simulink model "CabinGuard_MATLAB_simulation"  (R2024a)
settings: Solver=ode4  StartTime=0.0  StopTime=45  FixedStep=0.01  RelTol=1e-3
undefined symbols (not defined in the file or in its folder): ca_a_comf, ca_a_lo, ca_absvel, ca_clear, ca_d0, ca_det, ca_edge, ca_ego_id, ca_go_phase, ca_hw, ca_jdn, ca_jup, ca_kfeas, ca_lka_in, ca_lka_out, ca_lw0, ca_min_shift, ca_plant, ca_psi0, ca_pv, ca_sys, ca_t_act, ca_v0, ca_vlat, ca_wn, ca_X0, ca_Y0, driving, matlabshared
libraries: simulink x102, drivingscenarioandsensors x5, autolibshared x2, mpcadaslib x1, slpidlib x1
(part 3 of 4)

== system CabinGuard_MATLAB_simulation/GNC/Control ==
  d : Inport
  e2 : Inport  Port=2
  kappa : Inport  Port=3
  vmeas : Inport  Port=4
  yref : Inport  Port=5
  ydot : Inport  Port=6
  vref : Inport  Port=7
  aref : Inport  Port=8
  act : Inport  Port=9
  up : Inport  Port=10
  lo : Inport  Port=11
  DevErr : Sum  Inputs=+-
  FF : Sum
  GwClamp : simulink/Discontinuities/Saturation Dynamic  OutMin=[]  OutMax=[]  OutDataTypeStr=Inherit: Same as second input  OutDataType=fixdt(1, 16)  OutScaling=2^-10  DoSatur=off
  HoldA : Constant  Value=-1.5
  HoldAnd : Logic  AllPortsSameDT=off  OutDataTypeStr=boolean
  HoldSw : Switch  Criteria=u2 ~= 0  SaturateOnIntegerOverflow=off  InputSameDT=off
  InDev : Gain  Gain=ca_lka_in
  InKap : Gain  Gain=ca_lka_in
  InYaw : Gain  Gain=ca_lka_in
  LKA : mpcadaslib/Lane Keeping Assist System  ModelType=Use vehicle parameters  VehicleMass=1500  VehicleYawInertia=2500  LengthToFront=1.2  LengthToRear=1.5  FrontTireStiffness=98100  RearTireStiffness=78480  EgoModelMatrixA=[-4.4021 ,-12.4603;1.3913,-5.1868]  EgoModelMatrixB=[24.1270;15.8609]  EgoModelMatrixC=[1,0;0,1]  InitialLongVel=15  TransportLag=ca_lka_lag  MinSteering=-0.1  umin_ext=off  MaxSteering=0.1  umax_ext=off  Ts=0.1  PredictionHorizon=10  ControllerBehavior=ca_lka_beh  suboptimal=off  maxiter=10  datatypeopt=double  optmode=off  trackmode=off
  OutSt : Gain  Gain=ca_lka_out
  Slow : simulink/Logic and Bit Operations/Compare To Constant  relop=<  const=0.3  OutDataTypeStr=boolean
  SpeedPID : slpidlib/PID Controller  Controller=PI  Form=Parallel  TimeDomain=Discrete-time  UseExternalTs=off  SampleTime=0.1  IntegratorMethod=Forward Euler  FilterMethod=Forward Euler  ControllerParametersSource=internal  P=1.2  I=0.25  UseKiTs=off  D=0  UseExternalDerivativeSource=off  N=100  UseFilter=on  TunerSelectOption=Transfer Function Based (PID Tuner App)  InitialConditionSource=internal  InitialConditionForIntegrator=0  InitialConditionForFilter=0  DifferentiatorICPrevScaledInput=0  ExternalReset=none  TrackingMode=off  Kt=1  LimitOutput=on  SatLimitsSource=internal  UpperSaturationLimit=2  LowerSaturationLimit=-9  LinearizeAsGain=on  AntiWindupMode=clamping  Kb=1  LimitIntegrator=off  UpperIntegratorSaturationLimit=inf  LowerIntegratorSaturationLimit=-inf  POutMin=[]  POutMax=[]  IOutMin=[]  IOutMax=[]  DOutMin=[]  DOutMax=[]  NOutMin=[]  NOutMax=[]  SumOutMin=[]  SumOutMax=[]  SaturationOutMin=[]  SaturationOutMax=[]  PParamMin=[]  PParamMax=[]  IParamMin=[]  IParamMax=[]  DParamMin=[]  DParamMax=[]  NParamMin=[]  NParamMax=[]  KbParamMin=[]  KbParamMax=[]  KtParamMin=[]  KtParamMax=[]  KbOutMin=[]  KbOutMax=[]  KtOutMin=[]  KtOutMax=[]  IntegratorOutMin=[]  IntegratorOutMax=[]  FilterOutMin=[]  FilterOutMax=[]  SumI1OutMin=[]  SumI1OutMax=[]  SumI2OutMin=[]  SumI2OutMax=[]  SumI3OutMin=[]  SumI3OutMax=[]  SumI4OutMin=[]  SumI4OutMax=[]  SumDOutMin=[]  SumDOutMax=[]  DifferentiatorOutMin=[]  DifferentiatorOutMax=[]  FilterDiffOutCoefMin=[]  FilterDiffOutCoefMax=[]  ReciprocalOutMin=[]  ReciprocalOutMax=[]  SumDenOutMin=[]  SumDenOutMax=[]  SumNumOutMin=[]  SumNumOutMax=[]  DivideOutMin=[]  DivideOutMax=[]  UdiffTsProdOutMin=[]  UdiffTsProdOutMax=[]  NTsProdOutMin=[]  NTsProdOutMax=[]  UintegralTsProdOutMin=[]  UintegralTsProdOutMax=[]  UngainTsProdOutMin=[]  UngainTsProdOutMax=[]  ClampingZeroOutDataTypeStr=Inherit: Inherit via back propagation  ClampingZeroOutMin=[]  ClampingZeroOutMax=[]  FilterDenConstantOutDataTypeStr=Inherit: Inherit via back propagation  FilterDenConstantOutMin=[]  FilterDenConstantOutMax=[]  PCopyOutDataTypeStr=Inherit: Inherit via back propagation  PCopyOutMin=[]  PCopyOutMax=[]  NCopyOutDataTypeStr=Inherit: Inherit via back propagation  NCopyOutMin=[]  NCopyOutMax=[]  IntegratorContinuousStateAttributes=''  IntegratorStateMustResolveToSignalObject=off  IntegratorRTWStateStorageClass=Auto  FilterContinuousStateAttributes=''  FilterStateMustResolveToSignalObject=off  FilterRTWStateStorageClass=Auto  ParallelPVariant=InternalParameters  IdealPVariant=Disabled  IVariant=InternalParameters  DVariant=Disabled  IntegratorVariant=Discrete  SatVariant=Enabled  AWVariant=DiscClampingParallel  PCopyVariant=Disabled  TRVariant=Disabled  FdbkBlocksVariant=Forward  IdealPFdbkVariant=Disabled  SatFdbkVariant=Disabled  DerivativeFilterVariant=Disabled  NVariant=Disabled  NCopyVariant=Disabled_SignalSpec  FilterICVariant=Disabled  IntegratorICVariant=InternalICs  ExternalResetVariant=Disabled  TRSumVariant=Passthrough  SumFdbkVariant=Disabled  SumVariant=Sum_PI  TsampFilterVariant=InternalTs  TsampNgainVariant=Passthrough  TsampIntegralVariant=Disabled_SignalSpec  ExternalSaturationOutDataTypeStr=Inherit: Same as second input  DerivativeSourceVariant=Disabled
  StSw : Switch  Threshold=0.5  SaturateOnIntegerOverflow=off  InputSameDT=off
  SteerLim : Saturate  UpperLimit=0.1  LowerLimit=-0.1
  StraightC : Constant  Value=0
  VErr : Sum  Inputs=+-
  VLka : Saturate  UpperLimit=40  LowerLimit=1
  VxeS : Saturate  UpperLimit=inf  LowerLimit=2
  YawErr : Sum  Inputs=+-
  YdDivV : Product  Inputs=*/
  dcmd : Outport
  acmd : Outport  Port=2
  wires:
  vmeas/1 -> StSw/2, VLka/1, VErr/2, VxeS/1, Slow/1
  VErr/1 -> SpeedPID/1
  Slow/1 -> HoldAnd/2
  OutSt/1 -> SteerLim/1
  vref/1 -> VErr/1
  ydot/1 -> YdDivV/1
  VxeS/1 -> YdDivV/2
  act/1 -> HoldAnd/1
  d/1 -> DevErr/1
  yref/1 -> DevErr/2
  e2/1 -> YawErr/1
  YdDivV/1 -> YawErr/2
  InDev/1 -> LKA/3
  HoldAnd/1 -> HoldSw/2
  SpeedPID/1 -> FF/1
  aref/1 -> FF/2
  kappa/1 -> InKap/1
  StraightC/1 -> StSw/3
  DevErr/1 -> InDev/1
  SteerLim/1 -> StSw/1
  YawErr/1 -> InYaw/1
  up/1 -> GwClamp/1
  lo/1 -> GwClamp/3
  FF/1 -> GwClamp/2
  InKap/1 -> LKA/1
  VLka/1 -> LKA/2
  InYaw/1 -> LKA/4
  LKA/1 -> OutSt/1
  HoldA/1 -> HoldSw/1
  GwClamp/1 -> HoldSw/3
  HoldSw/1 -> acmd/1
  StSw/1 -> dcmd/1

== system CabinGuard_MATLAB_simulation/GNC/Decision ==
  areq : Inport
  occ : Inport  Port=2
  vmeas : Inport  Port=3
  go : Inport  Port=4
  ActDbl : DataTypeConversion  OutDataTypeStr=double  SaturateOnIntegerOverflow=off  RndMeth=Floor
  Active : DataTypeConversion  OutDataTypeStr=boolean  SaturateOnIntegerOverflow=off  RndMeth=Floor
  Clear : Constant  Value=ca_clear
  Comf : Constant  Value=ca_a_comf
  CommitD : UnitDelay  SampleTime=0.1  HasFrameUpgradeWarning=on
  CommitDbl : DataTypeConversion  OutDataTypeStr=double  SaturateOnIntegerOverflow=off  RndMeth=Floor
  CommitOr : Logic  Operator=OR  AllPortsSameDT=off  OutDataTypeStr=boolean
  Edge : Constant  Value=ca_edge
  FeasCmp : RelationalOperator  OutDataTypeStr=boolean  RndMeth=Simplest  InputSameDT=off
  FeasDiv : Product  Inputs=*/
  FeasK : Gain  Gain=ca_kfeas*ca_vlat
  Go : Logic  Inputs=4  AllPortsSameDT=off  OutDataTypeStr=boolean
  MaxA : MinMax  Function=max  Inputs=2
  NegA : Gain  Gain=-1
  NotOcc : Logic  Operator=NOT  AllPortsSameDT=off  OutDataTypeStr=boolean
  ReqScaled : Gain  Gain=1.25
  SatA : Saturate  UpperLimit=8.5  LowerLimit=0
  Space : simulink/Logic and Bit Operations/Compare To Constant  relop=>=  const=ca_min_shift  OutDataTypeStr=boolean
  UNeg : Gain  Gain=-1
  UProd : Product  Inputs=**
  YshT : Sum  Inputs=+-
  ulat : Outport
  adem : Outport  Port=2
  act : Outport  Port=3
  yshT : Outport  Port=4
  commit : Outport  Port=5
  wires:
  go/1 -> Active/1
  SatA/1 -> FeasDiv/2, NegA/1
  vmeas/1 -> FeasK/1
  areq/1 -> ReqScaled/1
  CommitDbl/1 -> UProd/1, commit/1
  Clear/1 -> YshT/1
  Comf/1 -> MaxA/1
  Edge/1 -> YshT/2
  FeasCmp/1 -> Go/4
  Space/1 -> Go/2
  MaxA/1 -> SatA/1
  CommitOr/1 -> CommitD/1, CommitDbl/1
  ReqScaled/1 -> MaxA/2
  FeasK/1 -> FeasDiv/1
  FeasDiv/1 -> FeasCmp/1
  NegA/1 -> adem/1
  occ/1 -> NotOcc/1
  YshT/1 -> UProd/2, Space/1, FeasCmp/2, yshT/1
  Active/1 -> Go/1, ActDbl/1
  NotOcc/1 -> Go/3
  ActDbl/1 -> act/1
  UNeg/1 -> ulat/1
  Go/1 -> CommitOr/1
  CommitD/1 -> CommitOr/2
  UProd/1 -> UNeg/1

== system CabinGuard_MATLAB_simulation/GNC/Guidance ==
  adem : Inport
  ulat : Inport  Port=2
  go : Inport  Port=3
  ASw : Switch  Criteria=u2 ~= 0  SaturateOnIntegerOverflow=off  InputSameDT=off
  AZero : Constant  Value=0
  ActD : DataTypeConversion  OutDataTypeStr=double  SaturateOnIntegerOverflow=off  RndMeth=Floor
  Active : DataTypeConversion  OutDataTypeStr=boolean  SaturateOnIntegerOverflow=off  RndMeth=Floor
  ClampMax : Constant  Value=ca_a_lo
  Jerk : RateLimiter  RisingSlewLimit=ca_jup  FallingSlewLimit=-ca_jdn  SampleTimeMode=inherited
  LatRL : RateLimiter  RisingSlewLimit=ca_vlat  FallingSlewLimit=-ca_vlat  SampleTimeMode=inherited
  LcY : TransferFcn  Numerator=ca_wn^2  Denominator=[1 2*ca_wn ca_wn^2]
  LcYd : TransferFcn  Numerator=[ca_wn^2 0]  Denominator=[1 2*ca_wn ca_wn^2]
  LoIdle : Constant  Value=-6
  LoMax : MinMax  Function=max  Inputs=2
  LoSw : Switch  Criteria=u2 ~= 0  SaturateOnIntegerOverflow=off  InputSameDT=off
  UpAct : Constant  Value=0
  UpIdle : Constant  Value=2
  UpSw : Switch  Criteria=u2 ~= 0  SaturateOnIntegerOverflow=off  InputSameDT=off
  VRef : Integrator  InitialCondition=ca_v0  LimitOutput=on  LowerSaturationLimit=0
  yref : Outport
  ydot : Outport  Port=2
  vref : Outport  Port=3
  aref : Outport  Port=4
  act : Outport  Port=5
  actd : Outport  Port=6
  up : Outport  Port=7
  lo : Outport  Port=8
  wires:
  go/1 -> Active/1
  adem/1 -> ASw/1, LoMax/2
  ulat/1 -> LatRL/1
  LoIdle/1 -> LoSw/3
  LoMax/1 -> LoSw/1
  LatRL/1 -> LcYd/1, LcY/1
  LoSw/1 -> lo/1
  ClampMax/1 -> LoMax/1
  ASw/1 -> Jerk/1
  Active/1 -> UpSw/2, ASw/2, act/1, ActD/1, LoSw/2
  AZero/1 -> ASw/3
  UpAct/1 -> UpSw/1
  UpIdle/1 -> UpSw/3
  UpSw/1 -> up/1
  LcY/1 -> yref/1
  VRef/1 -> vref/1
  LcYd/1 -> ydot/1
  ActD/1 -> actd/1
  Jerk/1 -> VRef/1, aref/1

== system CabinGuard_MATLAB_simulation/GNC/Navigation ==
  Lanes : Inport
  vx : Inport  Port=2
  B1 : BusSelector  OutputSignals=LateralOffset,HeadingAngle,Curvature
  B2 : BusSelector  OutputSignals=LateralOffset,HeadingAngle,Curvature
  DSum : Sum  Inputs=+-
  FinAbs : Abs  SaturateOnIntegerOverflow=off
  FinCmp : simulink/Logic and Bit Operations/Compare To Constant  relop=<  const=1000  OutDataTypeStr=boolean
  FinSum : Sum  Inputs=+++
  GoodAnd : Logic  AllPortsSameDT=off  OutDataTypeStr=boolean
  H{1..4} (4 alike) : Switch  Criteria=u2 ~= 0  SaturateOnIntegerOverflow=off  InputSameDT=off
  Hd1 : UnitDelay  SampleTime=0.1  HasFrameUpgradeWarning=on
  Hd2 : UnitDelay  SampleTime=0.1  HasFrameUpgradeWarning=on
  Hd3 : UnitDelay  SampleTime=0.1  HasFrameUpgradeWarning=on
  Hd4 : UnitDelay  InitialCondition=ca_lw0  SampleTime=0.1  HasFrameUpgradeWarning=on
  JDiv : Product  Inputs=*/
  JMul : Product  Inputs=**
  JRnd : Rounding  Operator=round
  Jump : Sum  Inputs=+-
  LBS : BusSelector  OutputSignals=LaneBoundaries,NumLaneBoundaries
  Lane1 : Selector  IndexOptions=Index vector (dialog)  Indices=1  OutputSizes=1
  Lane2 : Selector  IndexOptions=Index vector (dialog)  Indices=2  OutputSizes=1
  Nd : UnitDelay  SampleTime=0.1  HasFrameUpgradeWarning=on
  Nsum : Sum
  PrevE1 : UnitDelay  SampleTime=0.1  HasFrameUpgradeWarning=on
  Valid : simulink/Logic and Bit Operations/Compare To Constant  relop=>=  const=2  OutDataTypeStr=boolean
  WsNoise : RandomNumber  Variance=0.0025  Seed=7  SampleTime=0.1
  WsSum : Sum
  WsZoh : ZeroOrderHold  SampleTime=0.1
  gCv : Gain  Gain=0.5*pi/180
  gHd : Gain  Gain=-0.5*pi/180
  gOff : Gain  Gain=-0.5
  sCv : Sum
  sHd : Sum
  sOff : Sum
  sWd : Sum  Inputs=+-
  e1 : Outport
  e2 : Outport  Port=2
  kappa : Outport  Port=3
  vmeas : Outport  Port=4
  d : Outport  Port=5
  wires:
  Lanes/1 -> LBS/1
  vx/1 -> WsSum/1
  Valid/1 -> GoodAnd/1
  Lane1/1 -> B1/1
  gCv/1 -> H3/1, FinSum/3
  LBS/1 -> Lane1/1, Lane2/1  "<LaneBoundaries>"
  sCv/1 -> gCv/1
  WsSum/1 -> WsZoh/1
  gOff/1 -> H1/1, FinSum/1
  sWd/1 -> H4/1
  WsNoise/1 -> WsSum/2
  Jump/1 -> JDiv/1
  WsZoh/1 -> vmeas/1
  PrevE1/1 -> Jump/2
  LBS/2 -> Valid/1  "<NumLaneBoundaries>"
  Lane2/1 -> B2/1
  B1/1 -> sWd/1, sOff/1  "<LateralOffset>"
  B1/2 -> sHd/1  "<HeadingAngle>"
  B1/3 -> sCv/1  "<Curvature>"
  B2/1 -> sWd/2, sOff/2  "<LateralOffset>"
  H4/1 -> Hd4/1
  B2/2 -> sHd/2  "<HeadingAngle>"
  Hd3/1 -> H3/3
  B2/3 -> sCv/2  "<Curvature>"
  sOff/1 -> gOff/1
  Nsum/1 -> DSum/2, Nd/1
  sHd/1 -> gHd/1
  gHd/1 -> H2/1, FinSum/2
  FinSum/1 -> FinAbs/1
  JDiv/1 -> JRnd/1
  FinAbs/1 -> FinCmp/1
  H3/1 -> kappa/1, Hd3/1
  FinCmp/1 -> GoodAnd/2
  Hd1/1 -> H1/3
  JMul/1 -> Nsum/1
  Hd4/1 -> JDiv/2, JMul/2, H4/3
  GoodAnd/1 -> H3/2, H2/2, H4/2, H1/2
  H2/1 -> Hd2/1, e2/1
  Hd2/1 -> H2/3
  H1/1 -> Hd1/1, PrevE1/1, e1/1, DSum/1, Jump/1
  DSum/1 -> d/1
  Nd/1 -> Nsum/2
  JRnd/1 -> JMul/1

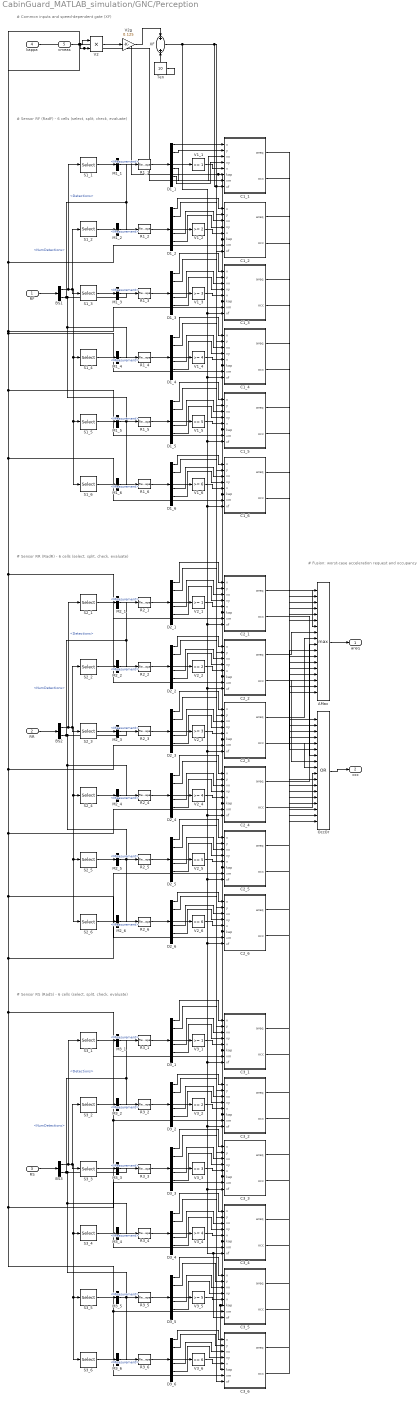
== system CabinGuard_MATLAB_simulation/GNC/Perception ==
  note: # Common inputs and speed-dependent gate (XF)
  note: # Sensor RF (RadF) - 6 cells (select, split, check, evaluate)
  note: # Sensor RR (RadR) - 6 cells (select, split, check, evaluate)
  note: # Sensor RS (RadS) - 6 cells (select, split, check, evaluate)
  note: # Fusion: worst-case acceleration request and occupancy
  RF : Inport
  RR : Inport  Port=2
  RS : Inport  Port=3
  kappa : Inport  Port=4
  vmeas : Inport  Port=5
  AMax : MinMax  Function=max  Inputs=18
  BS1 : BusSelector  OutputSignals=Detections,NumDetections
  BS2 : BusSelector  OutputSignals=Detections,NumDetections
  BS3 : BusSelector  OutputSignals=Detections,NumDetections
  C1_1 : Subsystem
  C1_2 : Subsystem
  C1_3 : Subsystem
  C1_4 : Subsystem
  C1_5 : Subsystem
  C1_6 : Subsystem
  C2_1 : Subsystem
  C2_2 : Subsystem
  C2_3 : Subsystem
  C2_4 : Subsystem
  C2_5 : Subsystem
  C2_6 : Subsystem
  C3_1 : Subsystem
  C3_2 : Subsystem
  C3_3 : Subsystem
  C3_4 : Subsystem
  C3_5 : Subsystem
  C3_6 : Subsystem
  D1_{1..6} (6 alike) : Demux  Outputs=6
  D2_{1..6} (6 alike) : Demux  Outputs=6
  D3_{1..6} (6 alike) : Demux  Outputs=6
  M1_{1..6} (6 alike) : BusSelector  OutputSignals=Measurement
  M2_{1..6} (6 alike) : BusSelector  OutputSignals=Measurement
  M3_{1..6} (6 alike) : BusSelector  OutputSignals=Measurement
  OccOr : Logic  Operator=OR  Inputs=18  AllPortsSameDT=off  OutDataTypeStr=boolean
  R1_{1..6} (6 alike) : Reshape
  R2_{1..6} (6 alike) : Reshape
  R3_{1..6} (6 alike) : Reshape
  S1_1 : Selector  IndexOptions=Index vector (dialog)  Indices=1  OutputSizes=1
  S1_2 : Selector  IndexOptions=Index vector (dialog)  Indices=2  OutputSizes=1
  S1_3 : Selector  IndexOptions=Index vector (dialog)  Indices=3  OutputSizes=1
  S1_4 : Selector  IndexOptions=Index vector (dialog)  Indices=4  OutputSizes=1
  S1_5 : Selector  IndexOptions=Index vector (dialog)  Indices=5  OutputSizes=1
  S1_6 : Selector  IndexOptions=Index vector (dialog)  Indices=6  OutputSizes=1
  S2_1 : Selector  IndexOptions=Index vector (dialog)  Indices=1  OutputSizes=1
  S2_2 : Selector  IndexOptions=Index vector (dialog)  Indices=2  OutputSizes=1
  S2_3 : Selector  IndexOptions=Index vector (dialog)  Indices=3  OutputSizes=1
  S2_4 : Selector  IndexOptions=Index vector (dialog)  Indices=4  OutputSizes=1
  S2_5 : Selector  IndexOptions=Index vector (dialog)  Indices=5  OutputSizes=1
  S2_6 : Selector  IndexOptions=Index vector (dialog)  Indices=6  OutputSizes=1
  S3_1 : Selector  IndexOptions=Index vector (dialog)  Indices=1  OutputSizes=1
  S3_2 : Selector  IndexOptions=Index vector (dialog)  Indices=2  OutputSizes=1
  S3_3 : Selector  IndexOptions=Index vector (dialog)  Indices=3  OutputSizes=1
  S3_4 : Selector  IndexOptions=Index vector (dialog)  Indices=4  OutputSizes=1
  S3_5 : Selector  IndexOptions=Index vector (dialog)  Indices=5  OutputSizes=1
  S3_6 : Selector  IndexOptions=Index vector (dialog)  Indices=6  OutputSizes=1
  Ten : Constant  Value=10
  V1_1 : simulink/Logic and Bit Operations/Compare To Constant  relop=>=  const=1  OutDataTypeStr=boolean
  V1_2 : simulink/Logic and Bit Operations/Compare To Constant  relop=>=  const=2  OutDataTypeStr=boolean
  V1_3 : simulink/Logic and Bit Operations/Compare To Constant  relop=>=  const=3  OutDataTypeStr=boolean
  V1_4 : simulink/Logic and Bit Operations/Compare To Constant  relop=>=  const=4  OutDataTypeStr=boolean
  V1_5 : simulink/Logic and Bit Operations/Compare To Constant  relop=>=  const=5  OutDataTypeStr=boolean
  V1_6 : simulink/Logic and Bit Operations/Compare To Constant  relop=>=  const=6  OutDataTypeStr=boolean
  V2 : Product  Inputs=**
  V2_1 : simulink/Logic and Bit Operations/Compare To Constant  relop=>=  const=1  OutDataTypeStr=boolean
  V2_2 : simulink/Logic and Bit Operations/Compare To Constant  relop=>=  const=2  OutDataTypeStr=boolean
  V2_3 : simulink/Logic and Bit Operations/Compare To Constant  relop=>=  const=3  OutDataTypeStr=boolean
  V2_4 : simulink/Logic and Bit Operations/Compare To Constant  relop=>=  const=4  OutDataTypeStr=boolean
  V2_5 : simulink/Logic and Bit Operations/Compare To Constant  relop=>=  const=5  OutDataTypeStr=boolean
  V2_6 : simulink/Logic and Bit Operations/Compare To Constant  relop=>=  const=6  OutDataTypeStr=boolean
  V2g : Gain  Gain=0.125
  V3_1 : simulink/Logic and Bit Operations/Compare To Constant  relop=>=  const=1  OutDataTypeStr=boolean
  V3_2 : simulink/Logic and Bit Operations/Compare To Constant  relop=>=  const=2  OutDataTypeStr=boolean
  V3_3 : simulink/Logic and Bit Operations/Compare To Constant  relop=>=  const=3  OutDataTypeStr=boolean
  V3_4 : simulink/Logic and Bit Operations/Compare To Constant  relop=>=  const=4  OutDataTypeStr=boolean
  V3_5 : simulink/Logic and Bit Operations/Compare To Constant  relop=>=  const=5  OutDataTypeStr=boolean
  V3_6 : simulink/Logic and Bit Operations/Compare To Constant  relop=>=  const=6  OutDataTypeStr=boolean
  XF : Sum
  areq : Outport
  occ : Outport  Port=2
  wires:
  vmeas/1 -> C3_5/7(vm), C3_6/7(vm), C3_3/7(vm), C3_1/7(vm), C2_5/7(vm), C2_4/7(vm), C2_3/7(vm), C2_1/7(vm), C1_5/7(vm), C1_3/7(vm), C1_2/7(vm), C1_1/7(vm), V2/2, V2/1, C3_2/7(vm), C3_4/7(vm), C2_6/7(vm), C2_2/7(vm), C1_6/7(vm), C1_4/7(vm)
  V2/1 -> V2g/1
  V2g/1 -> XF/1
  Ten/1 -> XF/2
  RF/1 -> BS1/1
  BS1/1 -> S1_2/1, S1_3/1, S1_4/1, S1_5/1, S1_6/1, S1_1/1  "<Detections>"
  S1_1/1 -> M1_1/1
  M1_1/1 -> R1_1/1  "<Measurement>"
  R1_1/1 -> D1_1/1
  BS1/2 -> V1_3/1, V1_5/1, V1_6/1, V1_4/1, V1_1/1, V1_2/1  "<NumDetections>"
  D1_1/1 -> C1_1/1(x)
  D1_1/2 -> C1_1/2(y)
  D1_1/4 -> C1_1/3(vx)
  D1_1/5 -> C1_1/4(vy)
  V1_1/1 -> C1_1/5(v)
  kappa/1 -> C3_6/6(kap), C3_5/6(kap), C3_4/6(kap), C3_3/6(kap), C3_2/6(kap), C3_1/6(kap), C2_6/6(kap), C2_5/6(kap), C2_4/6(kap), C2_3/6(kap), C2_2/6(kap), C2_1/6(kap), C1_6/6(kap), C1_5/6(kap), C1_4/6(kap), C1_3/6(kap), C1_2/6(kap), C1_1/6(kap)
  XF/1 -> C3_5/8(xf), C3_4/8(xf), C3_3/8(xf), C3_2/8(xf), C3_1/8(xf), C2_6/8(xf), C2_5/8(xf), C2_4/8(xf), C2_3/8(xf), C2_2/8(xf), C2_1/8(xf), C1_6/8(xf), C1_5/8(xf), C1_4/8(xf), C1_3/8(xf), C1_1/8(xf), C1_2/8(xf), C3_6/8(xf)
  C1_1/1(areq) -> AMax/1
  C1_1/2(occ) -> OccOr/1
  S1_2/1 -> M1_2/1
  M1_2/1 -> R1_2/1  "<Measurement>"
  R1_2/1 -> D1_2/1
  D1_2/1 -> C1_2/1(x)
  D1_2/2 -> C1_2/2(y)
  D1_2/4 -> C1_2/3(vx)
  D1_2/5 -> C1_2/4(vy)
  V1_2/1 -> C1_2/5(v)
  C1_2/1(areq) -> AMax/2
  C1_2/2(occ) -> OccOr/2
  S1_3/1 -> M1_3/1
  M1_3/1 -> R1_3/1  "<Measurement>"
  R1_3/1 -> D1_3/1
  D1_3/1 -> C1_3/1(x)
  D1_3/2 -> C1_3/2(y)
  D1_3/4 -> C1_3/3(vx)
  D1_3/5 -> C1_3/4(vy)
  V1_3/1 -> C1_3/5(v)
  C1_3/1(areq) -> AMax/3
  C1_3/2(occ) -> OccOr/3
  S1_4/1 -> M1_4/1
  M1_4/1 -> R1_4/1  "<Measurement>"
  R1_4/1 -> D1_4/1
  D1_4/1 -> C1_4/1(x)
  D1_4/2 -> C1_4/2(y)
  D1_4/4 -> C1_4/3(vx)
  D1_4/5 -> C1_4/4(vy)
  V1_4/1 -> C1_4/5(v)
  C1_4/1(areq) -> AMax/4
  C1_4/2(occ) -> OccOr/4
  S1_5/1 -> M1_5/1
  M1_5/1 -> R1_5/1  "<Measurement>"
  R1_5/1 -> D1_5/1
  D1_5/1 -> C1_5/1(x)
  D1_5/2 -> C1_5/2(y)
  D1_5/4 -> C1_5/3(vx)
  D1_5/5 -> C1_5/4(vy)
  V1_5/1 -> C1_5/5(v)
  C1_5/1(areq) -> AMax/5
  C1_5/2(occ) -> OccOr/5
  S1_6/1 -> M1_6/1
  M1_6/1 -> R1_6/1  "<Measurement>"
  R1_6/1 -> D1_6/1
  D1_6/1 -> C1_6/1(x)
  D1_6/2 -> C1_6/2(y)
  D1_6/4 -> C1_6/3(vx)
  D1_6/5 -> C1_6/4(vy)
  V1_6/1 -> C1_6/5(v)
  C1_6/1(areq) -> AMax/6
  C1_6/2(occ) -> OccOr/6
  RR/1 -> BS2/1
  BS2/1 -> S2_2/1, S2_3/1, S2_4/1, S2_5/1, S2_6/1, S2_1/1  "<Detections>"
  S2_1/1 -> M2_1/1
  M2_1/1 -> R2_1/1  "<Measurement>"
  R2_1/1 -> D2_1/1
  BS2/2 -> V2_3/1, V2_5/1, V2_6/1, V2_4/1, V2_1/1, V2_2/1  "<NumDetections>"
  D2_1/1 -> C2_1/1(x)
  D2_1/2 -> C2_1/2(y)
  D2_1/4 -> C2_1/3(vx)
  D2_1/5 -> C2_1/4(vy)
  V2_1/1 -> C2_1/5(v)
  C2_1/1(areq) -> AMax/7
  C2_1/2(occ) -> OccOr/7
  S2_2/1 -> M2_2/1
  M2_2/1 -> R2_2/1  "<Measurement>"
  R2_2/1 -> D2_2/1
  D2_2/1 -> C2_2/1(x)
  D2_2/2 -> C2_2/2(y)
  D2_2/4 -> C2_2/3(vx)
  D2_2/5 -> C2_2/4(vy)
  V2_2/1 -> C2_2/5(v)
  C2_2/1(areq) -> AMax/8
  C2_2/2(occ) -> OccOr/8
  S2_3/1 -> M2_3/1
  M2_3/1 -> R2_3/1  "<Measurement>"
  R2_3/1 -> D2_3/1
  D2_3/1 -> C2_3/1(x)
  D2_3/2 -> C2_3/2(y)
  D2_3/4 -> C2_3/3(vx)
  D2_3/5 -> C2_3/4(vy)
  V2_3/1 -> C2_3/5(v)
  C2_3/1(areq) -> AMax/9
  C2_3/2(occ) -> OccOr/9
  S2_4/1 -> M2_4/1
  M2_4/1 -> R2_4/1  "<Measurement>"
  R2_4/1 -> D2_4/1
  D2_4/1 -> C2_4/1(x)
  D2_4/2 -> C2_4/2(y)
  D2_4/4 -> C2_4/3(vx)
  D2_4/5 -> C2_4/4(vy)
  V2_4/1 -> C2_4/5(v)
  C2_4/1(areq) -> AMax/10
  C2_4/2(occ) -> OccOr/10
  S2_5/1 -> M2_5/1
  M2_5/1 -> R2_5/1  "<Measurement>"
  R2_5/1 -> D2_5/1
  D2_5/1 -> C2_5/1(x)
  D2_5/2 -> C2_5/2(y)
  D2_5/4 -> C2_5/3(vx)
  D2_5/5 -> C2_5/4(vy)
  V2_5/1 -> C2_5/5(v)
  C2_5/1(areq) -> AMax/11
  C2_5/2(occ) -> OccOr/11
  S2_6/1 -> M2_6/1
  M2_6/1 -> R2_6/1  "<Measurement>"
  R2_6/1 -> D2_6/1
  D2_6/1 -> C2_6/1(x)
  D2_6/2 -> C2_6/2(y)
  D2_6/4 -> C2_6/3(vx)
  D2_6/5 -> C2_6/4(vy)
  V2_6/1 -> C2_6/5(v)
  C2_6/1(areq) -> AMax/12
  C2_6/2(occ) -> OccOr/12
  RS/1 -> BS3/1
  BS3/1 -> S3_2/1, S3_3/1, S3_4/1, S3_5/1, S3_6/1, S3_1/1  "<Detections>"
  S3_1/1 -> M3_1/1
  M3_1/1 -> R3_1/1  "<Measurement>"
  R3_1/1 -> D3_1/1
  BS3/2 -> V3_3/1, V3_5/1, V3_6/1, V3_4/1, V3_1/1, V3_2/1  "<NumDetections>"
  D3_1/1 -> C3_1/1(x)
  D3_1/2 -> C3_1/2(y)
  D3_1/4 -> C3_1/3(vx)
  D3_1/5 -> C3_1/4(vy)
  V3_1/1 -> C3_1/5(v)
  C3_1/1(areq) -> AMax/13
  C3_1/2(occ) -> OccOr/13
  S3_2/1 -> M3_2/1
  M3_2/1 -> R3_2/1  "<Measurement>"
  R3_2/1 -> D3_2/1
  D3_2/1 -> C3_2/1(x)
  D3_2/2 -> C3_2/2(y)
  D3_2/4 -> C3_2/3(vx)
  D3_2/5 -> C3_2/4(vy)
  V3_2/1 -> C3_2/5(v)
  C3_2/1(areq) -> AMax/14
  C3_2/2(occ) -> OccOr/14
  S3_3/1 -> M3_3/1
  M3_3/1 -> R3_3/1  "<Measurement>"
  R3_3/1 -> D3_3/1
  D3_3/1 -> C3_3/1(x)
  D3_3/2 -> C3_3/2(y)
  D3_3/4 -> C3_3/3(vx)
  D3_3/5 -> C3_3/4(vy)
  V3_3/1 -> C3_3/5(v)
  C3_3/1(areq) -> AMax/15
  C3_3/2(occ) -> OccOr/15
  S3_4/1 -> M3_4/1
  M3_4/1 -> R3_4/1  "<Measurement>"
  R3_4/1 -> D3_4/1
  D3_4/1 -> C3_4/1(x)
  D3_4/2 -> C3_4/2(y)
  D3_4/4 -> C3_4/3(vx)
  D3_4/5 -> C3_4/4(vy)
  V3_4/1 -> C3_4/5(v)
  C3_4/1(areq) -> AMax/16
  C3_4/2(occ) -> OccOr/16
  S3_5/1 -> M3_5/1
  M3_5/1 -> R3_5/1  "<Measurement>"
  R3_5/1 -> D3_5/1
  D3_5/1 -> C3_5/1(x)
  D3_5/2 -> C3_5/2(y)
  D3_5/4 -> C3_5/3(vx)
  D3_5/5 -> C3_5/4(vy)
  V3_5/1 -> C3_5/5(v)
  C3_5/1(areq) -> AMax/17
  C3_5/2(occ) -> OccOr/17
  S3_6/1 -> M3_6/1
  M3_6/1 -> R3_6/1  "<Measurement>"
  R3_6/1 -> D3_6/1
  D3_6/1 -> C3_6/1(x)
  D3_6/2 -> C3_6/2(y)
  D3_6/4 -> C3_6/3(vx)
  D3_6/5 -> C3_6/4(vy)
  V3_6/1 -> C3_6/5(v)
  C3_6/1(areq) -> AMax/18
  C3_6/2(occ) -> OccOr/18
  AMax/1 -> areq/1
  OccOr/1 -> occ/1

== system CabinGuard_MATLAB_simulation/Vehicle/LBody ==
  FwF : Inport
  FwR : Inport  Port=2
  Grade : Inport  Port=3
  Wind : Inport  Port=4
  HoldIn : Inport  Port=5
  Brk : simulink/Logic and Bit Operations/Compare To Constant  relop=>  const=0.5  OutDataTypeStr=boolean
  CF : Constant  Value=4087.5
  CR : Constant  Value=3270
  Fsum : Sum
  HAnd : Logic  AllPortsSameDT=off  OutDataTypeStr=boolean
  HSw : Switch  Criteria=u2 ~= 0  SaturateOnIntegerOverflow=off  InputSameDT=off
  Hold : Gain  Gain=-20
  InvM : Gain  Gain=0.0006666666667
  Ix : Integrator  InitialCondition=ca_v0  LimitOutput=on  LowerSaturationLimit=0
  Kd : Gain  Gain=0.42175
  KhF : Gain  Gain=-152.7777778
  KhR : Gain  Gain=152.7777778
  Net : Sum  Inputs=+-
  Pitch : TransferFcn  Numerator=1  Denominator=[0.15 1]
  SF : Sum
  SR : Sum
  Slow : simulink/Logic and Bit Operations/Compare To Constant  relop=<  const=0.4  OutDataTypeStr=boolean
  TG : Terminator
  TW : Terminator
  V2 : Product
  Z : Constant  Value=0
  Info : Outport
  xdot : Outport  Port=2
  FzF : Outport  Port=3
  FzR : Outport  Port=4
  wires:
  Kd/1 -> Net/2
  V2/1 -> Kd/1
  HoldIn/1 -> Brk/1
  Grade/1 -> TG/1
  Slow/1 -> HAnd/1
  FwF/1 -> Fsum/1
  Wind/1 -> TW/1
  Z/1 -> Info/1
  InvM/1 -> HSw/3, Pitch/1
  FwR/1 -> Fsum/2
  Fsum/1 -> Net/1
  KhF/1 -> SF/1
  Brk/1 -> HAnd/2
  Net/1 -> InvM/1
  Ix/1 -> V2/1, Slow/1, Hold/1, xdot/1, V2/2
  HAnd/1 -> HSw/2
  Hold/1 -> HSw/1
  Pitch/1 -> KhF/1, KhR/1
  HSw/1 -> Ix/1
  CR/1 -> SR/2
  KhR/1 -> SR/1
  CF/1 -> SF/2
  SR/1 -> FzR/1
  SF/1 -> FzF/1

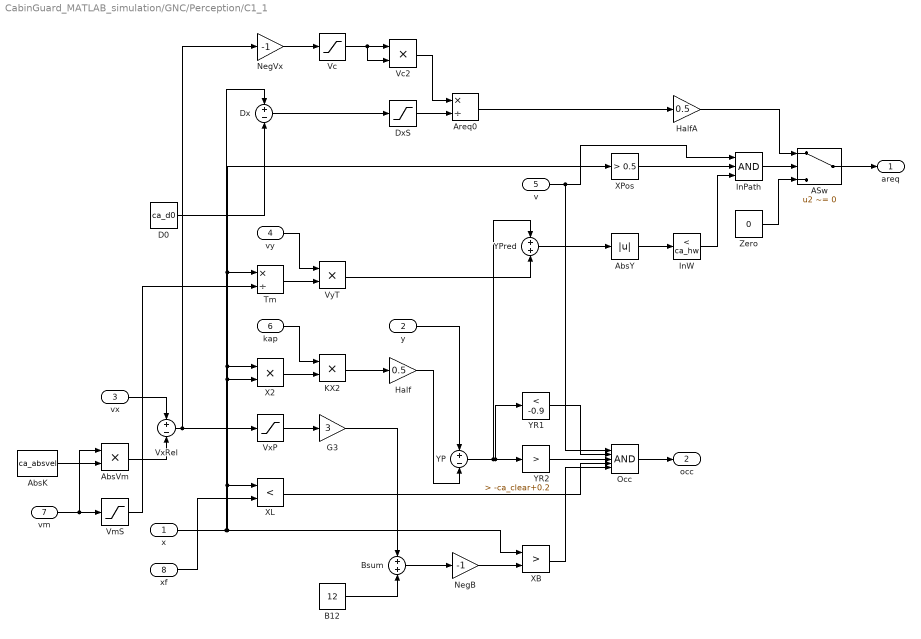
== system CabinGuard_MATLAB_simulation/GNC/Perception/C1_1 ==
  x : Inport
  y : Inport  Port=2
  vx : Inport  Port=3
  vy : Inport  Port=4
  v : Inport  Port=5
  kap : Inport  Port=6
  vm : Inport  Port=7
  xf : Inport  Port=8
  ASw : Switch  Criteria=u2 ~= 0  SaturateOnIntegerOverflow=off  InputSameDT=off
  AbsK : Constant  Value=ca_absvel
  AbsVm : Product  Inputs=**
  AbsY : Abs  SaturateOnIntegerOverflow=off
  Areq0 : Product  Inputs=*/
  B12 : Constant  Value=12
  Bsum : Sum
  D0 : Constant  Value=ca_d0
  Dx : Sum  Inputs=+-
  DxS : Saturate  UpperLimit=inf  LowerLimit=0.5
  G3 : Gain  Gain=3
  Half : Gain  Gain=0.5
  HalfA : Gain  Gain=0.5
  InPath : Logic  Inputs=3  AllPortsSameDT=off  OutDataTypeStr=boolean
  InW : simulink/Logic and Bit Operations/Compare To Constant  relop=<  const=ca_hw  OutDataTypeStr=boolean
  KX2 : Product  Inputs=**
  NegB : Gain  Gain=-1
  NegVx : Gain  Gain=-1
  Occ : Logic  Inputs=5  AllPortsSameDT=off  OutDataTypeStr=boolean
  Tm : Product  Inputs=*/
  Vc : Saturate  UpperLimit=inf  LowerLimit=0
  Vc2 : Product  Inputs=**
  VmS : Saturate  UpperLimit=inf  LowerLimit=1
  VxP : Saturate  UpperLimit=inf  LowerLimit=0
  VxRel : Sum  Inputs=+-
  VyT : Product  Inputs=**
  X2 : Product  Inputs=**
  XB : RelationalOperator  Operator=>  OutDataTypeStr=boolean  RndMeth=Simplest  InputSameDT=off
  XL : RelationalOperator  Operator=<  OutDataTypeStr=boolean  RndMeth=Simplest  InputSameDT=off
  XPos : simulink/Logic and Bit Operations/Compare To Constant  relop=>  const=0.5  OutDataTypeStr=boolean
  YP : Sum  Inputs=+-
  YPred : Sum
  YR1 : simulink/Logic and Bit Operations/Compare To Constant  relop=<  const=-0.9  OutDataTypeStr=boolean
  YR2 : simulink/Logic and Bit Operations/Compare To Constant  relop=>  const=-ca_clear+0.2  OutDataTypeStr=boolean
  Zero : Constant  Value=0
  areq : Outport
  occ : Outport  Port=2
  wires:
  Tm/1 -> VyT/2
  AbsK/1 -> AbsVm/2
  vx/1 -> VxRel/1
  InPath/1 -> ASw/2
  vm/1 -> AbsVm/1, VmS/1
  AbsVm/1 -> VxRel/2
  NegB/1 -> XB/2
  VmS/1 -> Tm/2
  x/1 -> Tm/1, XPos/1, X2/1, X2/2, XL/1, XB/1, Dx/1
  D0/1 -> Dx/2
  VxRel/1 -> VxP/1, NegVx/1
  Bsum/1 -> NegB/1
  xf/1 -> XL/2
  VxP/1 -> G3/1
  kap/1 -> KX2/1
  NegVx/1 -> Vc/1
  Dx/1 -> DxS/1
  vy/1 -> VyT/1
  X2/1 -> KX2/2
  XL/1 -> Occ/4
  InW/1 -> InPath/3
  Vc/1 -> Vc2/2, Vc2/1
  VyT/1 -> YPred/2
  AbsY/1 -> InW/1
  Vc2/1 -> Areq0/1
  KX2/1 -> Half/1
  y/1 -> YP/1
  G3/1 -> Bsum/1
  B12/1 -> Bsum/2
  DxS/1 -> Areq0/2
  Half/1 -> YP/2
  Areq0/1 -> HalfA/1
  YP/1 -> YR2/1, YR1/1, YPred/1
  HalfA/1 -> ASw/1
  v/1 -> InPath/1, Occ/1
  YPred/1 -> AbsY/1
  YR1/1 -> Occ/2
  YR2/1 -> Occ/3
  XB/1 -> Occ/5
  XPos/1 -> InPath/2
  Occ/1 -> occ/1
  Zero/1 -> ASw/3
  ASw/1 -> areq/1

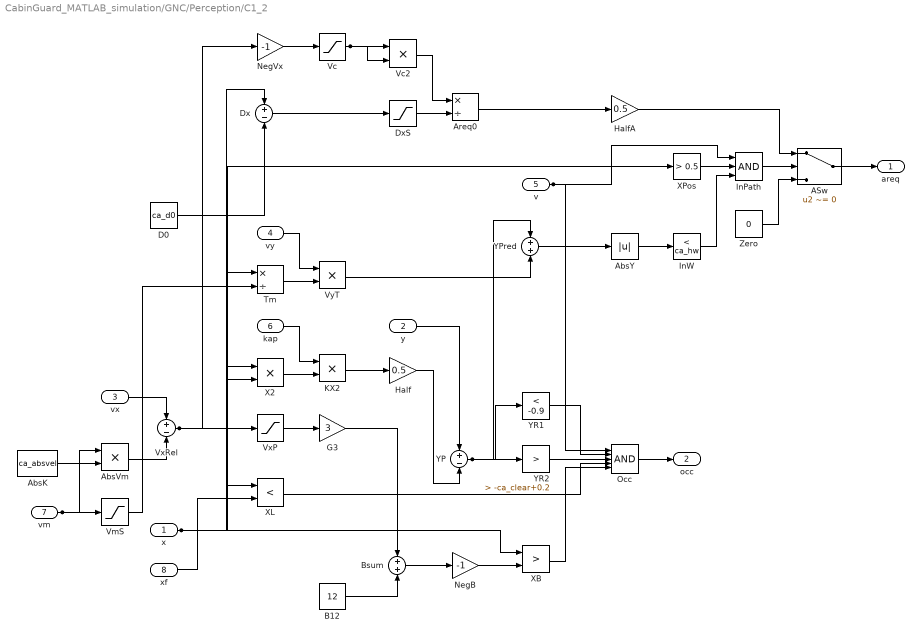
== system CabinGuard_MATLAB_simulation/GNC/Perception/C1_2 ==
  x : Inport
  y : Inport  Port=2
  vx : Inport  Port=3
  vy : Inport  Port=4
  v : Inport  Port=5
  kap : Inport  Port=6
  vm : Inport  Port=7
  xf : Inport  Port=8
  ASw : Switch  Criteria=u2 ~= 0  SaturateOnIntegerOverflow=off  InputSameDT=off
  AbsK : Constant  Value=ca_absvel
  AbsVm : Product  Inputs=**
  AbsY : Abs  SaturateOnIntegerOverflow=off
  Areq0 : Product  Inputs=*/
  B12 : Constant  Value=12
  Bsum : Sum
  D0 : Constant  Value=ca_d0
  Dx : Sum  Inputs=+-
  DxS : Saturate  UpperLimit=inf  LowerLimit=0.5
  G3 : Gain  Gain=3
  Half : Gain  Gain=0.5
  HalfA : Gain  Gain=0.5
  InPath : Logic  Inputs=3  AllPortsSameDT=off  OutDataTypeStr=boolean
  InW : simulink/Logic and Bit Operations/Compare To Constant  relop=<  const=ca_hw  OutDataTypeStr=boolean
  KX2 : Product  Inputs=**
  NegB : Gain  Gain=-1
  NegVx : Gain  Gain=-1
  Occ : Logic  Inputs=5  AllPortsSameDT=off  OutDataTypeStr=boolean
  Tm : Product  Inputs=*/
  Vc : Saturate  UpperLimit=inf  LowerLimit=0
  Vc2 : Product  Inputs=**
  VmS : Saturate  UpperLimit=inf  LowerLimit=1
  VxP : Saturate  UpperLimit=inf  LowerLimit=0
  VxRel : Sum  Inputs=+-
  VyT : Product  Inputs=**
  X2 : Product  Inputs=**
  XB : RelationalOperator  Operator=>  OutDataTypeStr=boolean  RndMeth=Simplest  InputSameDT=off
  XL : RelationalOperator  Operator=<  OutDataTypeStr=boolean  RndMeth=Simplest  InputSameDT=off
  XPos : simulink/Logic and Bit Operations/Compare To Constant  relop=>  const=0.5  OutDataTypeStr=boolean
  YP : Sum  Inputs=+-
  YPred : Sum
  YR1 : simulink/Logic and Bit Operations/Compare To Constant  relop=<  const=-0.9  OutDataTypeStr=boolean
  YR2 : simulink/Logic and Bit Operations/Compare To Constant  relop=>  const=-ca_clear+0.2  OutDataTypeStr=boolean
  Zero : Constant  Value=0
  areq : Outport
  occ : Outport  Port=2
  wires:
  AbsK/1 -> AbsVm/2
  Zero/1 -> ASw/3
  Areq0/1 -> HalfA/1
  D0/1 -> Dx/2
  HalfA/1 -> ASw/1
  YPred/1 -> AbsY/1
  vx/1 -> VxRel/1
  AbsVm/1 -> VxRel/2
  vm/1 -> AbsVm/1, VmS/1
  VmS/1 -> Tm/2
  xf/1 -> XL/2
  VxRel/1 -> VxP/1, NegVx/1
  AbsY/1 -> InW/1
  x/1 -> XB/1, XPos/1, XL/1, Tm/1, Dx/1, X2/2, X2/1
  G3/1 -> Bsum/1
  NegVx/1 -> Vc/1
  InPath/1 -> ASw/2
  Dx/1 -> DxS/1
  vy/1 -> VyT/1
  Tm/1 -> VyT/2
  kap/1 -> KX2/1
  Occ/1 -> occ/1
  X2/1 -> KX2/2
  VxP/1 -> G3/1
  XL/1 -> Occ/4
  Vc/1 -> Vc2/2, Vc2/1
  VyT/1 -> YPred/2
  KX2/1 -> Half/1
  B12/1 -> Bsum/2
  Vc2/1 -> Areq0/1
  NegB/1 -> XB/2
  y/1 -> YP/1
  DxS/1 -> Areq0/2
  Half/1 -> YP/2
  Bsum/1 -> NegB/1
  YP/1 -> YPred/1, YR1/1, YR2/1
  v/1 -> InPath/1, Occ/1
  YR1/1 -> Occ/2
  YR2/1 -> Occ/3
  XB/1 -> Occ/5
  XPos/1 -> InPath/2
  InW/1 -> InPath/3
  ASw/1 -> areq/1

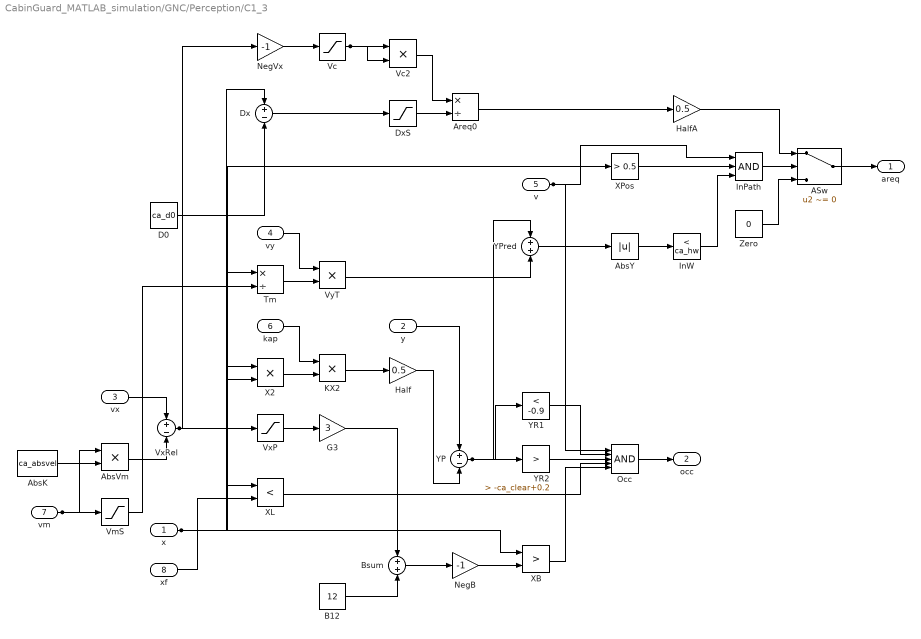
== system CabinGuard_MATLAB_simulation/GNC/Perception/C1_3 ==
  x : Inport
  y : Inport  Port=2
  vx : Inport  Port=3
  vy : Inport  Port=4
  v : Inport  Port=5
  kap : Inport  Port=6
  vm : Inport  Port=7
  xf : Inport  Port=8
  ASw : Switch  Criteria=u2 ~= 0  SaturateOnIntegerOverflow=off  InputSameDT=off
  AbsK : Constant  Value=ca_absvel
  AbsVm : Product  Inputs=**
  AbsY : Abs  SaturateOnIntegerOverflow=off
  Areq0 : Product  Inputs=*/
  B12 : Constant  Value=12
  Bsum : Sum
  D0 : Constant  Value=ca_d0
  Dx : Sum  Inputs=+-
  DxS : Saturate  UpperLimit=inf  LowerLimit=0.5
  G3 : Gain  Gain=3
  Half : Gain  Gain=0.5
  HalfA : Gain  Gain=0.5
  InPath : Logic  Inputs=3  AllPortsSameDT=off  OutDataTypeStr=boolean
  InW : simulink/Logic and Bit Operations/Compare To Constant  relop=<  const=ca_hw  OutDataTypeStr=boolean
  KX2 : Product  Inputs=**
  NegB : Gain  Gain=-1
  NegVx : Gain  Gain=-1
  Occ : Logic  Inputs=5  AllPortsSameDT=off  OutDataTypeStr=boolean
  Tm : Product  Inputs=*/
  Vc : Saturate  UpperLimit=inf  LowerLimit=0
  Vc2 : Product  Inputs=**
  VmS : Saturate  UpperLimit=inf  LowerLimit=1
  VxP : Saturate  UpperLimit=inf  LowerLimit=0
  VxRel : Sum  Inputs=+-
  VyT : Product  Inputs=**
  X2 : Product  Inputs=**
  XB : RelationalOperator  Operator=>  OutDataTypeStr=boolean  RndMeth=Simplest  InputSameDT=off
  XL : RelationalOperator  Operator=<  OutDataTypeStr=boolean  RndMeth=Simplest  InputSameDT=off
  XPos : simulink/Logic and Bit Operations/Compare To Constant  relop=>  const=0.5  OutDataTypeStr=boolean
  YP : Sum  Inputs=+-
  YPred : Sum
  YR1 : simulink/Logic and Bit Operations/Compare To Constant  relop=<  const=-0.9  OutDataTypeStr=boolean
  YR2 : simulink/Logic and Bit Operations/Compare To Constant  relop=>  const=-ca_clear+0.2  OutDataTypeStr=boolean
  Zero : Constant  Value=0
  areq : Outport
  occ : Outport  Port=2
  wires:
  AbsK/1 -> AbsVm/2
  AbsY/1 -> InW/1
  vx/1 -> VxRel/1
  vm/1 -> AbsVm/1, VmS/1
  AbsVm/1 -> VxRel/2
  VmS/1 -> Tm/2
  x/1 -> XB/1, XPos/1, Tm/1, Dx/1, X2/2, XL/1, X2/1
  D0/1 -> Dx/2
  VxRel/1 -> VxP/1, NegVx/1
  Bsum/1 -> NegB/1
  xf/1 -> XL/2
  NegVx/1 -> Vc/1
  YR1/1 -> Occ/2
  Dx/1 -> DxS/1
  vy/1 -> VyT/1
  Tm/1 -> VyT/2
  XB/1 -> Occ/5
  kap/1 -> KX2/1
  X2/1 -> KX2/2
  VxP/1 -> G3/1
  XL/1 -> Occ/4
  Vc/1 -> Vc2/2, Vc2/1
  VyT/1 -> YPred/2
  KX2/1 -> Half/1
  y/1 -> YP/1
  G3/1 -> Bsum/1
  B12/1 -> Bsum/2
  Vc2/1 -> Areq0/1
  DxS/1 -> Areq0/2
  Half/1 -> YP/2
  Areq0/1 -> HalfA/1
  YP/1 -> YPred/1, YR2/1, YR1/1
  NegB/1 -> XB/2
  HalfA/1 -> ASw/1
  v/1 -> InPath/1, Occ/1
  YPred/1 -> AbsY/1
  YR2/1 -> Occ/3
  XPos/1 -> InPath/2
  Occ/1 -> occ/1
  InW/1 -> InPath/3
  InPath/1 -> ASw/2
  Zero/1 -> ASw/3
  ASw/1 -> areq/1

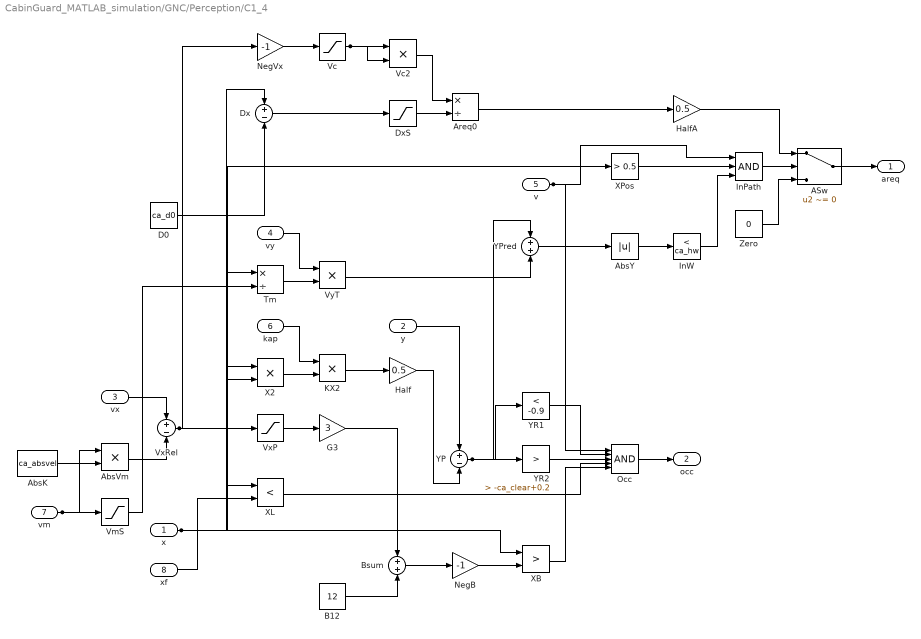
== system CabinGuard_MATLAB_simulation/GNC/Perception/C1_4 ==
  x : Inport
  y : Inport  Port=2
  vx : Inport  Port=3
  vy : Inport  Port=4
  v : Inport  Port=5
  kap : Inport  Port=6
  vm : Inport  Port=7
  xf : Inport  Port=8
  ASw : Switch  Criteria=u2 ~= 0  SaturateOnIntegerOverflow=off  InputSameDT=off
  AbsK : Constant  Value=ca_absvel
  AbsVm : Product  Inputs=**
  AbsY : Abs  SaturateOnIntegerOverflow=off
  Areq0 : Product  Inputs=*/
  B12 : Constant  Value=12
  Bsum : Sum
  D0 : Constant  Value=ca_d0
  Dx : Sum  Inputs=+-
  DxS : Saturate  UpperLimit=inf  LowerLimit=0.5
  G3 : Gain  Gain=3
  Half : Gain  Gain=0.5
  HalfA : Gain  Gain=0.5
  InPath : Logic  Inputs=3  AllPortsSameDT=off  OutDataTypeStr=boolean
  InW : simulink/Logic and Bit Operations/Compare To Constant  relop=<  const=ca_hw  OutDataTypeStr=boolean
  KX2 : Product  Inputs=**
  NegB : Gain  Gain=-1
  NegVx : Gain  Gain=-1
  Occ : Logic  Inputs=5  AllPortsSameDT=off  OutDataTypeStr=boolean
  Tm : Product  Inputs=*/
  Vc : Saturate  UpperLimit=inf  LowerLimit=0
  Vc2 : Product  Inputs=**
  VmS : Saturate  UpperLimit=inf  LowerLimit=1
  VxP : Saturate  UpperLimit=inf  LowerLimit=0
  VxRel : Sum  Inputs=+-
  VyT : Product  Inputs=**
  X2 : Product  Inputs=**
  XB : RelationalOperator  Operator=>  OutDataTypeStr=boolean  RndMeth=Simplest  InputSameDT=off
  XL : RelationalOperator  Operator=<  OutDataTypeStr=boolean  RndMeth=Simplest  InputSameDT=off
  XPos : simulink/Logic and Bit Operations/Compare To Constant  relop=>  const=0.5  OutDataTypeStr=boolean
  YP : Sum  Inputs=+-
  YPred : Sum
  YR1 : simulink/Logic and Bit Operations/Compare To Constant  relop=<  const=-0.9  OutDataTypeStr=boolean
  YR2 : simulink/Logic and Bit Operations/Compare To Constant  relop=>  const=-ca_clear+0.2  OutDataTypeStr=boolean
  Zero : Constant  Value=0
  areq : Outport
  occ : Outport  Port=2
  wires:
  AbsK/1 -> AbsVm/2
  vx/1 -> VxRel/1
  vm/1 -> VmS/1, AbsVm/1
  Zero/1 -> ASw/3
  AbsVm/1 -> VxRel/2
  VmS/1 -> Tm/2
  v/1 -> InPath/1, Occ/1
  Vc/1 -> Vc2/2, Vc2/1
  x/1 -> Dx/1, Tm/1, XB/1, X2/2, XL/1, X2/1, XPos/1
  D0/1 -> Dx/2
  Bsum/1 -> NegB/1
  XL/1 -> Occ/4
  VxRel/1 -> VxP/1, NegVx/1
  xf/1 -> XL/2
  NegVx/1 -> Vc/1
  YR1/1 -> Occ/2
  Dx/1 -> DxS/1
  vy/1 -> VyT/1
  Tm/1 -> VyT/2
  kap/1 -> KX2/1
  X2/1 -> KX2/2
  XB/1 -> Occ/5
  B12/1 -> Bsum/2
  G3/1 -> Bsum/1
  VxP/1 -> G3/1
  VyT/1 -> YPred/2
  KX2/1 -> Half/1
  AbsY/1 -> InW/1
  Vc2/1 -> Areq0/1
  DxS/1 -> Areq0/2
  y/1 -> YP/1
  YP/1 -> YR2/1, YR1/1, YPred/1
  Half/1 -> YP/2
  Areq0/1 -> HalfA/1
  YR2/1 -> Occ/3
  NegB/1 -> XB/2
  YPred/1 -> AbsY/1
  XPos/1 -> InPath/2
  Occ/1 -> occ/1
  HalfA/1 -> ASw/1
  InW/1 -> InPath/3
  InPath/1 -> ASw/2
  ASw/1 -> areq/1

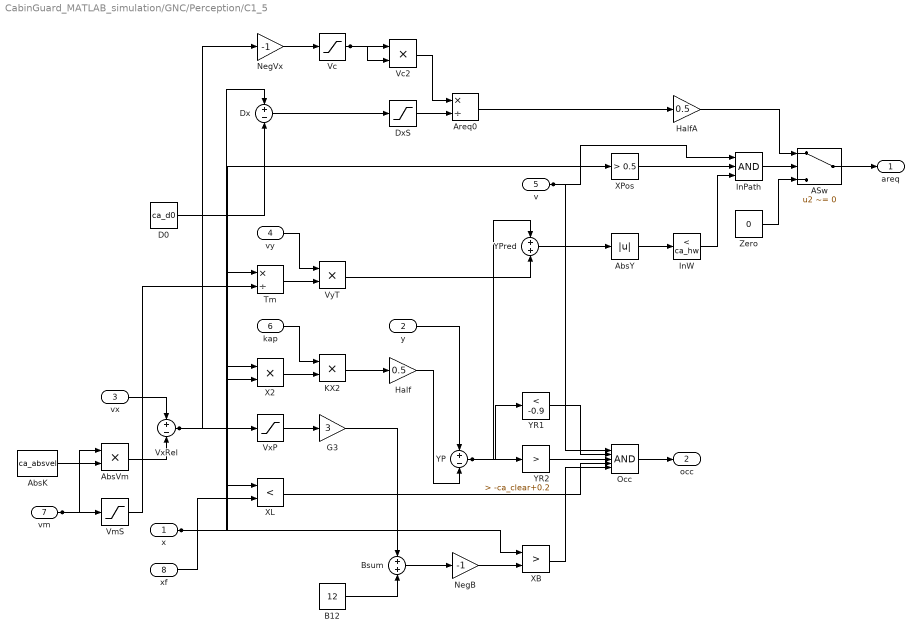
== system CabinGuard_MATLAB_simulation/GNC/Perception/C1_5 ==
  x : Inport
  y : Inport  Port=2
  vx : Inport  Port=3
  vy : Inport  Port=4
  v : Inport  Port=5
  kap : Inport  Port=6
  vm : Inport  Port=7
  xf : Inport  Port=8
  ASw : Switch  Criteria=u2 ~= 0  SaturateOnIntegerOverflow=off  InputSameDT=off
  AbsK : Constant  Value=ca_absvel
  AbsVm : Product  Inputs=**
  AbsY : Abs  SaturateOnIntegerOverflow=off
  Areq0 : Product  Inputs=*/
  B12 : Constant  Value=12
  Bsum : Sum
  D0 : Constant  Value=ca_d0
  Dx : Sum  Inputs=+-
  DxS : Saturate  UpperLimit=inf  LowerLimit=0.5
  G3 : Gain  Gain=3
  Half : Gain  Gain=0.5
  HalfA : Gain  Gain=0.5
  InPath : Logic  Inputs=3  AllPortsSameDT=off  OutDataTypeStr=boolean
  InW : simulink/Logic and Bit Operations/Compare To Constant  relop=<  const=ca_hw  OutDataTypeStr=boolean
  KX2 : Product  Inputs=**
  NegB : Gain  Gain=-1
  NegVx : Gain  Gain=-1
  Occ : Logic  Inputs=5  AllPortsSameDT=off  OutDataTypeStr=boolean
  Tm : Product  Inputs=*/
  Vc : Saturate  UpperLimit=inf  LowerLimit=0
  Vc2 : Product  Inputs=**
  VmS : Saturate  UpperLimit=inf  LowerLimit=1
  VxP : Saturate  UpperLimit=inf  LowerLimit=0
  VxRel : Sum  Inputs=+-
  VyT : Product  Inputs=**
  X2 : Product  Inputs=**
  XB : RelationalOperator  Operator=>  OutDataTypeStr=boolean  RndMeth=Simplest  InputSameDT=off
  XL : RelationalOperator  Operator=<  OutDataTypeStr=boolean  RndMeth=Simplest  InputSameDT=off
  XPos : simulink/Logic and Bit Operations/Compare To Constant  relop=>  const=0.5  OutDataTypeStr=boolean
  YP : Sum  Inputs=+-
  YPred : Sum
  YR1 : simulink/Logic and Bit Operations/Compare To Constant  relop=<  const=-0.9  OutDataTypeStr=boolean
  YR2 : simulink/Logic and Bit Operations/Compare To Constant  relop=>  const=-ca_clear+0.2  OutDataTypeStr=boolean
  Zero : Constant  Value=0
  areq : Outport
  occ : Outport  Port=2
  wires:
  AbsK/1 -> AbsVm/2
  Bsum/1 -> NegB/1
  XL/1 -> Occ/4
  VxRel/1 -> VxP/1, NegVx/1
  vx/1 -> VxRel/1
  vm/1 -> AbsVm/1, VmS/1
  AbsVm/1 -> VxRel/2
  NegB/1 -> XB/2
  VmS/1 -> Tm/2
  InW/1 -> InPath/3
  D0/1 -> Dx/2
  NegVx/1 -> Vc/1
  x/1 -> XPos/1, Dx/1, XL/1, X2/2, X2/1, Tm/1, XB/1
  Vc2/1 -> Areq0/1
  xf/1 -> XL/2
  YR1/1 -> Occ/2
  Dx/1 -> DxS/1
  KX2/1 -> Half/1
  vy/1 -> VyT/1
  Tm/1 -> VyT/2
  kap/1 -> KX2/1
  Occ/1 -> occ/1
  X2/1 -> KX2/2
  VxP/1 -> G3/1
  Vc/1 -> Vc2/2, Vc2/1
  VyT/1 -> YPred/2
  G3/1 -> Bsum/1
  B12/1 -> Bsum/2
  DxS/1 -> Areq0/2
  y/1 -> YP/1
  Half/1 -> YP/2
  Areq0/1 -> HalfA/1
  YP/1 -> YR2/1, YR1/1, YPred/1
  XB/1 -> Occ/5
  v/1 -> InPath/1, Occ/1
  YPred/1 -> AbsY/1
  ASw/1 -> areq/1
  YR2/1 -> Occ/3
  XPos/1 -> InPath/2
  AbsY/1 -> InW/1
  HalfA/1 -> ASw/1
  InPath/1 -> ASw/2
  Zero/1 -> ASw/3

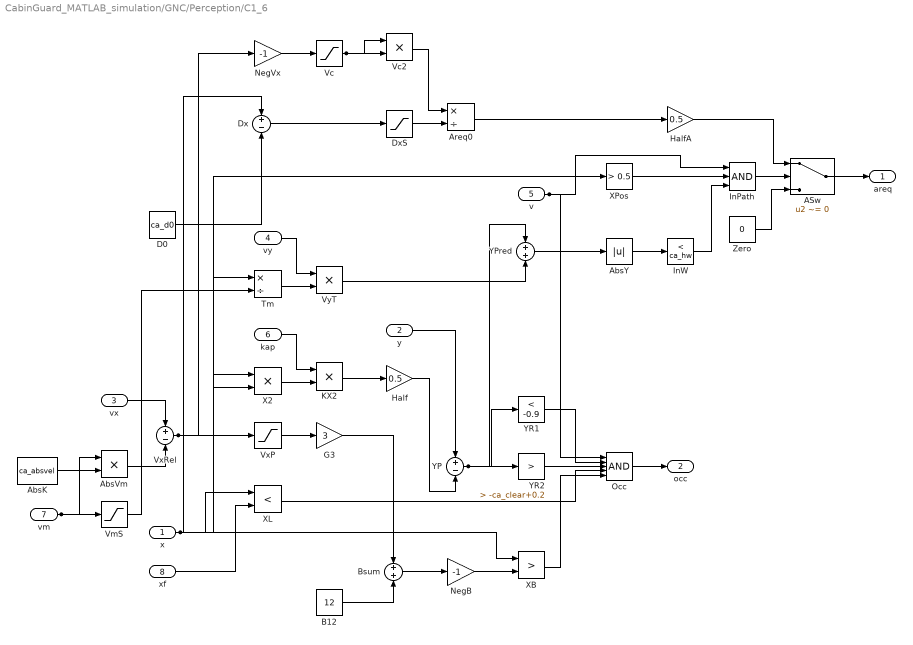
== system CabinGuard_MATLAB_simulation/GNC/Perception/C1_6 ==
  x : Inport
  y : Inport  Port=2
  vx : Inport  Port=3
  vy : Inport  Port=4
  v : Inport  Port=5
  kap : Inport  Port=6
  vm : Inport  Port=7
  xf : Inport  Port=8
  ASw : Switch  Criteria=u2 ~= 0  SaturateOnIntegerOverflow=off  InputSameDT=off
  AbsK : Constant  Value=ca_absvel
  AbsVm : Product  Inputs=**
  AbsY : Abs  SaturateOnIntegerOverflow=off
  Areq0 : Product  Inputs=*/
  B12 : Constant  Value=12
  Bsum : Sum
  D0 : Constant  Value=ca_d0
  Dx : Sum  Inputs=+-
  DxS : Saturate  UpperLimit=inf  LowerLimit=0.5
  G3 : Gain  Gain=3
  Half : Gain  Gain=0.5
  HalfA : Gain  Gain=0.5
  InPath : Logic  Inputs=3  AllPortsSameDT=off  OutDataTypeStr=boolean
  InW : simulink/Logic and Bit Operations/Compare To Constant  relop=<  const=ca_hw  OutDataTypeStr=boolean
  KX2 : Product  Inputs=**
  NegB : Gain  Gain=-1
  NegVx : Gain  Gain=-1
  Occ : Logic  Inputs=5  AllPortsSameDT=off  OutDataTypeStr=boolean
  Tm : Product  Inputs=*/
  Vc : Saturate  UpperLimit=inf  LowerLimit=0
  Vc2 : Product  Inputs=**
  VmS : Saturate  UpperLimit=inf  LowerLimit=1
  VxP : Saturate  UpperLimit=inf  LowerLimit=0
  VxRel : Sum  Inputs=+-
  VyT : Product  Inputs=**
  X2 : Product  Inputs=**
  XB : RelationalOperator  Operator=>  OutDataTypeStr=boolean  RndMeth=Simplest  InputSameDT=off
  XL : RelationalOperator  Operator=<  OutDataTypeStr=boolean  RndMeth=Simplest  InputSameDT=off
  XPos : simulink/Logic and Bit Operations/Compare To Constant  relop=>  const=0.5  OutDataTypeStr=boolean
  YP : Sum  Inputs=+-
  YPred : Sum
  YR1 : simulink/Logic and Bit Operations/Compare To Constant  relop=<  const=-0.9  OutDataTypeStr=boolean
  YR2 : simulink/Logic and Bit Operations/Compare To Constant  relop=>  const=-ca_clear+0.2  OutDataTypeStr=boolean
  Zero : Constant  Value=0
  areq : Outport
  occ : Outport  Port=2
  wires:
  VxP/1 -> G3/1
  AbsK/1 -> AbsVm/2
  VmS/1 -> Tm/2
  vx/1 -> VxRel/1
  YR2/1 -> Occ/3
  NegB/1 -> XB/2
  vm/1 -> AbsVm/1, VmS/1
  VxRel/1 -> VxP/1, NegVx/1
  AbsVm/1 -> VxRel/2
  D0/1 -> Dx/2
  v/1 -> InPath/1, Occ/1
  x/1 -> Dx/1, XB/1, Tm/1, XPos/1, X2/1, X2/2, XL/1
  xf/1 -> XL/2
  NegVx/1 -> Vc/1
  Dx/1 -> DxS/1
  YPred/1 -> AbsY/1
  vy/1 -> VyT/1
  Tm/1 -> VyT/2
  B12/1 -> Bsum/2
  kap/1 -> KX2/1
  X2/1 -> KX2/2
  Occ/1 -> occ/1
  XL/1 -> Occ/4
  Vc/1 -> Vc2/1, Vc2/2
  VyT/1 -> YPred/2
  KX2/1 -> Half/1
  XB/1 -> Occ/5
  G3/1 -> Bsum/1
  YR1/1 -> Occ/2
  Vc2/1 -> Areq0/1
  DxS/1 -> Areq0/2
  y/1 -> YP/1
  Half/1 -> YP/2
  Bsum/1 -> NegB/1
  Areq0/1 -> HalfA/1
  YP/1 -> YPred/1, YR2/1, YR1/1
  Zero/1 -> ASw/3
  XPos/1 -> InPath/2
  AbsY/1 -> InW/1
  HalfA/1 -> ASw/1
  InW/1 -> InPath/3
  InPath/1 -> ASw/2
  ASw/1 -> areq/1

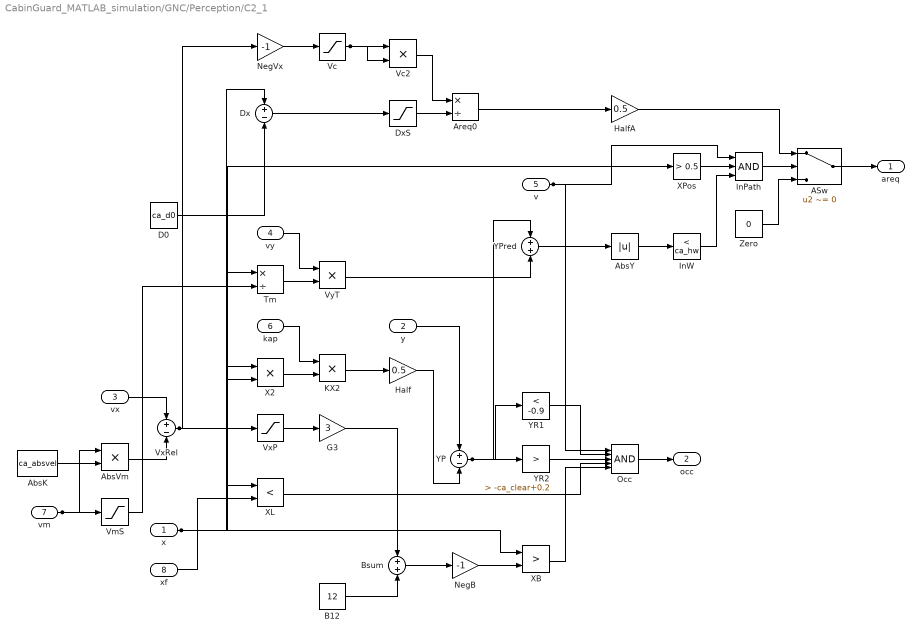
== system CabinGuard_MATLAB_simulation/GNC/Perception/C2_1 ==
  x : Inport
  y : Inport  Port=2
  vx : Inport  Port=3
  vy : Inport  Port=4
  v : Inport  Port=5
  kap : Inport  Port=6
  vm : Inport  Port=7
  xf : Inport  Port=8
  ASw : Switch  Criteria=u2 ~= 0  SaturateOnIntegerOverflow=off  InputSameDT=off
  AbsK : Constant  Value=ca_absvel
  AbsVm : Product  Inputs=**
  AbsY : Abs  SaturateOnIntegerOverflow=off
  Areq0 : Product  Inputs=*/
  B12 : Constant  Value=12
  Bsum : Sum
  D0 : Constant  Value=ca_d0
  Dx : Sum  Inputs=+-
  DxS : Saturate  UpperLimit=inf  LowerLimit=0.5
  G3 : Gain  Gain=3
  Half : Gain  Gain=0.5
  HalfA : Gain  Gain=0.5
  InPath : Logic  Inputs=3  AllPortsSameDT=off  OutDataTypeStr=boolean
  InW : simulink/Logic and Bit Operations/Compare To Constant  relop=<  const=ca_hw  OutDataTypeStr=boolean
  KX2 : Product  Inputs=**
  NegB : Gain  Gain=-1
  NegVx : Gain  Gain=-1
  Occ : Logic  Inputs=5  AllPortsSameDT=off  OutDataTypeStr=boolean
  Tm : Product  Inputs=*/
  Vc : Saturate  UpperLimit=inf  LowerLimit=0
  Vc2 : Product  Inputs=**
  VmS : Saturate  UpperLimit=inf  LowerLimit=1
  VxP : Saturate  UpperLimit=inf  LowerLimit=0
  VxRel : Sum  Inputs=+-
  VyT : Product  Inputs=**
  X2 : Product  Inputs=**
  XB : RelationalOperator  Operator=>  OutDataTypeStr=boolean  RndMeth=Simplest  InputSameDT=off
  XL : RelationalOperator  Operator=<  OutDataTypeStr=boolean  RndMeth=Simplest  InputSameDT=off
  XPos : simulink/Logic and Bit Operations/Compare To Constant  relop=>  const=0.5  OutDataTypeStr=boolean
  YP : Sum  Inputs=+-
  YPred : Sum
  YR1 : simulink/Logic and Bit Operations/Compare To Constant  relop=<  const=-0.9  OutDataTypeStr=boolean
  YR2 : simulink/Logic and Bit Operations/Compare To Constant  relop=>  const=-ca_clear+0.2  OutDataTypeStr=boolean
  Zero : Constant  Value=0
  areq : Outport
  occ : Outport  Port=2
  wires:
  AbsK/1 -> AbsVm/2
  InPath/1 -> ASw/2
  VmS/1 -> Tm/2
  KX2/1 -> Half/1
  vx/1 -> VxRel/1
  vm/1 -> AbsVm/1, VmS/1
  AbsVm/1 -> VxRel/2
  x/1 -> XB/1, XPos/1, XL/1, Tm/1, X2/2, Dx/1, X2/1
  Vc/1 -> Vc2/2, Vc2/1
  D0/1 -> Dx/2
  VxRel/1 -> VxP/1, NegVx/1
  Occ/1 -> occ/1
  xf/1 -> XL/2
  B12/1 -> Bsum/2
  kap/1 -> KX2/1
  NegVx/1 -> Vc/1
  Dx/1 -> DxS/1
  YR1/1 -> Occ/2
  vy/1 -> VyT/1
  DxS/1 -> Areq0/2
  Tm/1 -> VyT/2
  X2/1 -> KX2/2
  VxP/1 -> G3/1
  XL/1 -> Occ/4
  VyT/1 -> YPred/2
  G3/1 -> Bsum/1
  Vc2/1 -> Areq0/1
  y/1 -> YP/1
  Half/1 -> YP/2
  Bsum/1 -> NegB/1
  Areq0/1 -> HalfA/1
  YP/1 -> YPred/1, YR2/1, YR1/1
  NegB/1 -> XB/2
  YR2/1 -> Occ/3
  v/1 -> InPath/1, Occ/1
  YPred/1 -> AbsY/1
  Zero/1 -> ASw/3
  XB/1 -> Occ/5
  HalfA/1 -> ASw/1
  AbsY/1 -> InW/1
  XPos/1 -> InPath/2
  InW/1 -> InPath/3
  ASw/1 -> areq/1

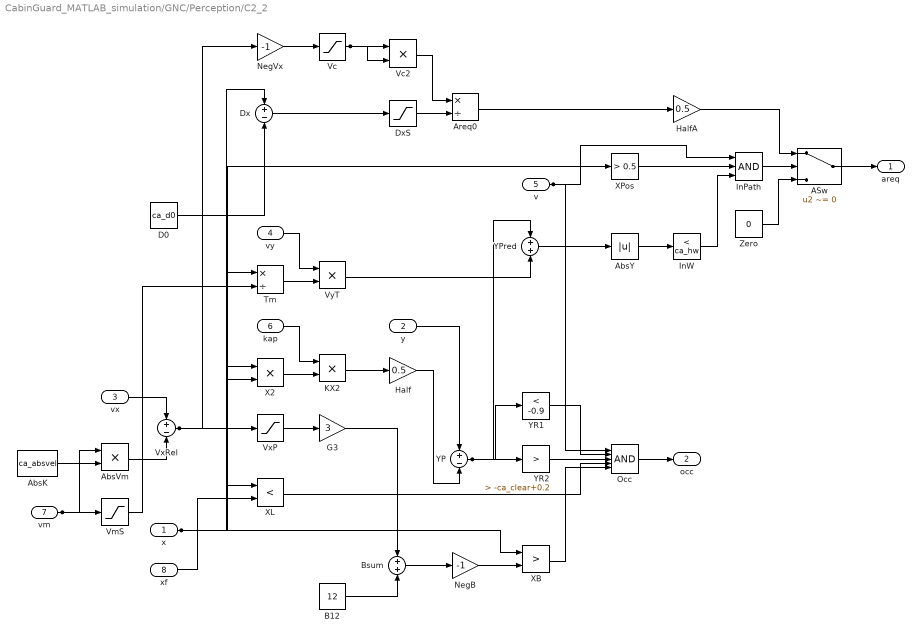
== system CabinGuard_MATLAB_simulation/GNC/Perception/C2_2 ==
  x : Inport
  y : Inport  Port=2
  vx : Inport  Port=3
  vy : Inport  Port=4
  v : Inport  Port=5
  kap : Inport  Port=6
  vm : Inport  Port=7
  xf : Inport  Port=8
  ASw : Switch  Criteria=u2 ~= 0  SaturateOnIntegerOverflow=off  InputSameDT=off
  AbsK : Constant  Value=ca_absvel
  AbsVm : Product  Inputs=**
  AbsY : Abs  SaturateOnIntegerOverflow=off
  Areq0 : Product  Inputs=*/
  B12 : Constant  Value=12
  Bsum : Sum
  D0 : Constant  Value=ca_d0
  Dx : Sum  Inputs=+-
  DxS : Saturate  UpperLimit=inf  LowerLimit=0.5
  G3 : Gain  Gain=3
  Half : Gain  Gain=0.5
  HalfA : Gain  Gain=0.5
  InPath : Logic  Inputs=3  AllPortsSameDT=off  OutDataTypeStr=boolean
  InW : simulink/Logic and Bit Operations/Compare To Constant  relop=<  const=ca_hw  OutDataTypeStr=boolean
  KX2 : Product  Inputs=**
  NegB : Gain  Gain=-1
  NegVx : Gain  Gain=-1
  Occ : Logic  Inputs=5  AllPortsSameDT=off  OutDataTypeStr=boolean
  Tm : Product  Inputs=*/
  Vc : Saturate  UpperLimit=inf  LowerLimit=0
  Vc2 : Product  Inputs=**
  VmS : Saturate  UpperLimit=inf  LowerLimit=1
  VxP : Saturate  UpperLimit=inf  LowerLimit=0
  VxRel : Sum  Inputs=+-
  VyT : Product  Inputs=**
  X2 : Product  Inputs=**
  XB : RelationalOperator  Operator=>  OutDataTypeStr=boolean  RndMeth=Simplest  InputSameDT=off
  XL : RelationalOperator  Operator=<  OutDataTypeStr=boolean  RndMeth=Simplest  InputSameDT=off
  XPos : simulink/Logic and Bit Operations/Compare To Constant  relop=>  const=0.5  OutDataTypeStr=boolean
  YP : Sum  Inputs=+-
  YPred : Sum
  YR1 : simulink/Logic and Bit Operations/Compare To Constant  relop=<  const=-0.9  OutDataTypeStr=boolean
  YR2 : simulink/Logic and Bit Operations/Compare To Constant  relop=>  const=-ca_clear+0.2  OutDataTypeStr=boolean
  Zero : Constant  Value=0
  areq : Outport
  occ : Outport  Port=2
  wires:
  KX2/1 -> Half/1
  AbsK/1 -> AbsVm/2
  AbsY/1 -> InW/1
  vx/1 -> VxRel/1
  InPath/1 -> ASw/2
  vm/1 -> VmS/1, AbsVm/1
  XPos/1 -> InPath/2
  D0/1 -> Dx/2
  AbsVm/1 -> VxRel/2
  vy/1 -> VyT/1
  VmS/1 -> Tm/2
  VxRel/1 -> VxP/1, NegVx/1
  InW/1 -> InPath/3
  x/1 -> XB/1, XPos/1, Dx/1, Tm/1, X2/2, X2/1, XL/1
  YR2/1 -> Occ/3
  xf/1 -> XL/2
  ASw/1 -> areq/1
  y/1 -> YP/1
  NegVx/1 -> Vc/1
  Dx/1 -> DxS/1
  Tm/1 -> VyT/2
  kap/1 -> KX2/1
  X2/1 -> KX2/2
  VxP/1 -> G3/1
  XL/1 -> Occ/4
  Vc/1 -> Vc2/2, Vc2/1
  VyT/1 -> YPred/2
  G3/1 -> Bsum/1
  B12/1 -> Bsum/2
  Vc2/1 -> Areq0/1
  DxS/1 -> Areq0/2
  Half/1 -> YP/2
  Bsum/1 -> NegB/1
  Areq0/1 -> HalfA/1
  YP/1 -> YPred/1, YR2/1, YR1/1
  NegB/1 -> XB/2
  v/1 -> InPath/1, Occ/1
  YPred/1 -> AbsY/1
  YR1/1 -> Occ/2
  XB/1 -> Occ/5
  Occ/1 -> occ/1
  HalfA/1 -> ASw/1
  Zero/1 -> ASw/3

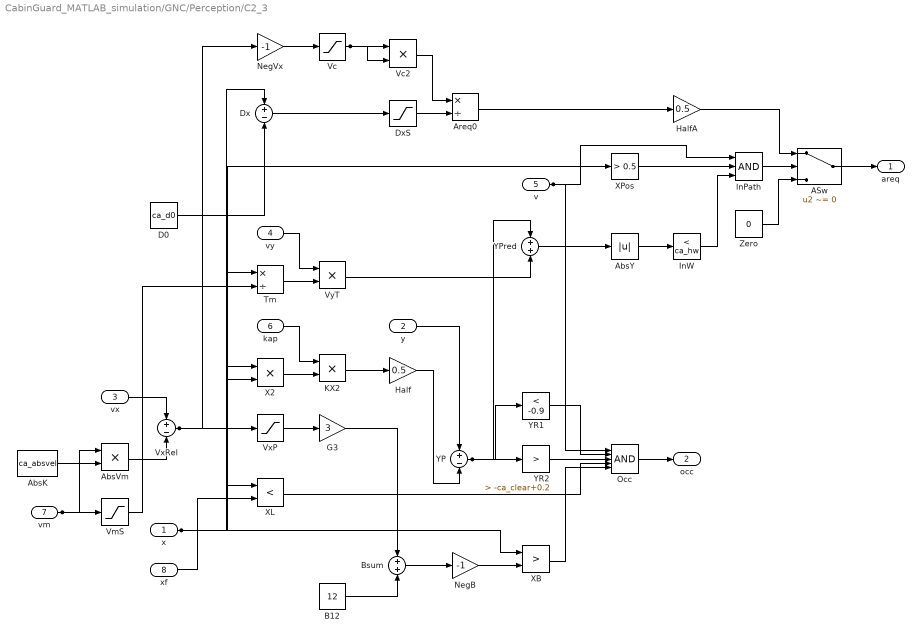
== system CabinGuard_MATLAB_simulation/GNC/Perception/C2_3 ==
  x : Inport
  y : Inport  Port=2
  vx : Inport  Port=3
  vy : Inport  Port=4
  v : Inport  Port=5
  kap : Inport  Port=6
  vm : Inport  Port=7
  xf : Inport  Port=8
  ASw : Switch  Criteria=u2 ~= 0  SaturateOnIntegerOverflow=off  InputSameDT=off
  AbsK : Constant  Value=ca_absvel
  AbsVm : Product  Inputs=**
  AbsY : Abs  SaturateOnIntegerOverflow=off
  Areq0 : Product  Inputs=*/
  B12 : Constant  Value=12
  Bsum : Sum
  D0 : Constant  Value=ca_d0
  Dx : Sum  Inputs=+-
  DxS : Saturate  UpperLimit=inf  LowerLimit=0.5
  G3 : Gain  Gain=3
  Half : Gain  Gain=0.5
  HalfA : Gain  Gain=0.5
  InPath : Logic  Inputs=3  AllPortsSameDT=off  OutDataTypeStr=boolean
  InW : simulink/Logic and Bit Operations/Compare To Constant  relop=<  const=ca_hw  OutDataTypeStr=boolean
  KX2 : Product  Inputs=**
  NegB : Gain  Gain=-1
  NegVx : Gain  Gain=-1
  Occ : Logic  Inputs=5  AllPortsSameDT=off  OutDataTypeStr=boolean
  Tm : Product  Inputs=*/
  Vc : Saturate  UpperLimit=inf  LowerLimit=0
  Vc2 : Product  Inputs=**
  VmS : Saturate  UpperLimit=inf  LowerLimit=1
  VxP : Saturate  UpperLimit=inf  LowerLimit=0
  VxRel : Sum  Inputs=+-
  VyT : Product  Inputs=**
  X2 : Product  Inputs=**
  XB : RelationalOperator  Operator=>  OutDataTypeStr=boolean  RndMeth=Simplest  InputSameDT=off
  XL : RelationalOperator  Operator=<  OutDataTypeStr=boolean  RndMeth=Simplest  InputSameDT=off
  XPos : simulink/Logic and Bit Operations/Compare To Constant  relop=>  const=0.5  OutDataTypeStr=boolean
  YP : Sum  Inputs=+-
  YPred : Sum
  YR1 : simulink/Logic and Bit Operations/Compare To Constant  relop=<  const=-0.9  OutDataTypeStr=boolean
  YR2 : simulink/Logic and Bit Operations/Compare To Constant  relop=>  const=-ca_clear+0.2  OutDataTypeStr=boolean
  Zero : Constant  Value=0
  areq : Outport
  occ : Outport  Port=2
  wires:
  X2/1 -> KX2/2
  vy/1 -> VyT/1
  VxRel/1 -> NegVx/1, VxP/1
  AbsK/1 -> AbsVm/2
  InPath/1 -> ASw/2
  vm/1 -> AbsVm/1, VmS/1
  vx/1 -> VxRel/1
  NegVx/1 -> Vc/1
  AbsVm/1 -> VxRel/2
  x/1 -> XL/1, X2/2, XPos/1, Dx/1, X2/1, Tm/1, XB/1
  VmS/1 -> Tm/2
  D0/1 -> Dx/2
  xf/1 -> XL/2
  Dx/1 -> DxS/1
  Tm/1 -> VyT/2
  kap/1 -> KX2/1
  G3/1 -> Bsum/1
  VxP/1 -> G3/1
  XL/1 -> Occ/4
  InW/1 -> InPath/3
  Vc/1 -> Vc2/2, Vc2/1
  VyT/1 -> YPred/2
  KX2/1 -> Half/1
  B12/1 -> Bsum/2
  Vc2/1 -> Areq0/1
  DxS/1 -> Areq0/2
  y/1 -> YP/1
  Half/1 -> YP/2
  Bsum/1 -> NegB/1
  Areq0/1 -> HalfA/1
  YP/1 -> YPred/1, YR2/1, YR1/1
  NegB/1 -> XB/2
  v/1 -> InPath/1, Occ/1
  YPred/1 -> AbsY/1
  YR1/1 -> Occ/2
  YR2/1 -> Occ/3
  XB/1 -> Occ/5
  XPos/1 -> InPath/2
  AbsY/1 -> InW/1
  Occ/1 -> occ/1
  HalfA/1 -> ASw/1
  Zero/1 -> ASw/3
  ASw/1 -> areq/1
